simulink library "actuators_lib"  (R2018b)
settings: Solver=VariableStepAuto  StartTime=0.0  StopTime=10.0  RelTol=1e-3
libraries: $bdroot x1
settings Model: Creator=Ybeyer  LastModifiedBy=yannic
settings DebuggingCC: LibraryContextMissingDiagnostic=none
settings SFSimCC: SimUseLocalCustomCode=off
settings RTWCC: RTWUseLocalCustomCode=off
settings CodeAppCC: StateflowObjectComments=on

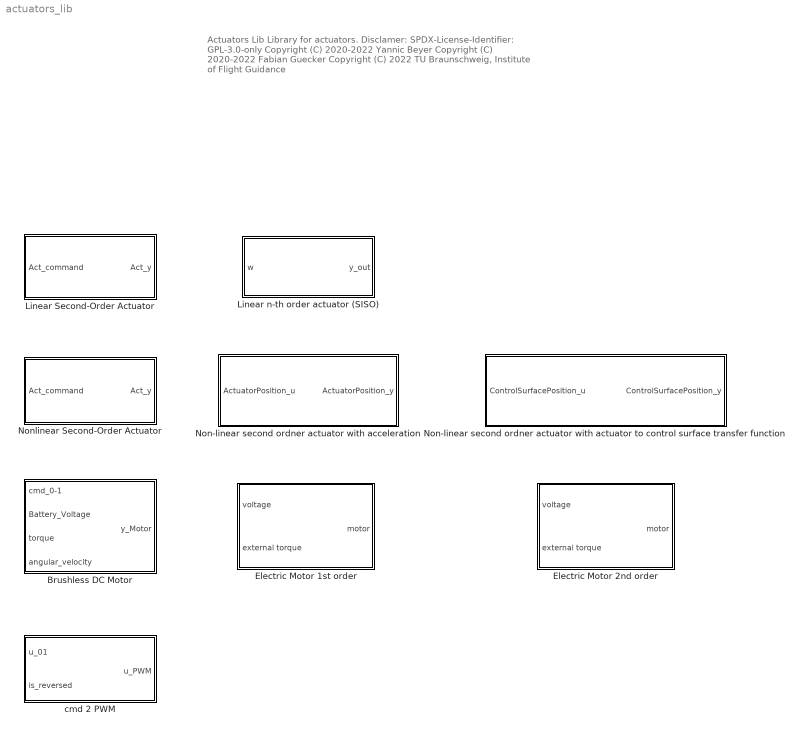
== system actuators_lib ==
  note: Actuators Lib
      |
      | Library for actuators.
      |
      | Disclamer:
      | SPDX-License-Identifier: GPL-3.0-only
      |
      | Copyright (C) 2020-2022 Yannic Beyer
      | Copyright (C) 2020-2022 Fabian Guecker
      | Copyright (C) 2022 TU Braunschweig, Institute of Flight Guidance
  Brushless DC Motor : Subsystem  mask{K_T=30/pi/920, J_prop=1e-04, R_i=0.042, IC_omega=0, omega_max=Inf, omega_min=0}
      mask prompts: K_T "Motor torque constant, Nm/A"; J_prop "Motor moment of inertia, kg-m^2"; R_i "Motor internal resistance, Ohm"; IC_omega "Initial motor angular velocity, 1/s"; omega_max "Maximum motor angular velocity, 1/s"; omega_min "Minimum motor angular velocity, 1/s"
      mask DialogControl DescGroupVar Prompt: Brushless DC Motor
      mask DialogControl DescTextVar Prompt: First-Order Brushless Direct Current Motor model.
      mask DialogControl Control3 Prompt: Inputs:
      mask DialogControl Control4 Prompt: Command (cmd_0-1, -)
      mask DialogControl Control5 Prompt: Battery Voltage, V
      mask DialogControl Control6 Prompt: torque, Nm
      mask DialogControl Control8 Prompt: Outputs:
      mask DialogControl Control9 Prompt: angular velocity (omega, 1/s)
      mask DialogControl Control10 Prompt: angular acceleration (dot_omega, 1/s^2)
  Electric Motor 1st order : Subsystem  mask{K_T=30/pi/920, J_prop=1e-04, R_i=0.042, IC_omega=0, omega_max=Inf, omega_min=0}
      mask prompts: K_T "Motor torque constant, Nm/A"; J_prop "Motor moment of inertia, kg-m^2"; R_i "Motor internal resistance, Ohm"; IC_omega "Initial motor angular velocity, rad/s"; omega_max "Maximum motor angular velocity, rad/s"; omega_min "Minimum motor angular velocity, rad/s"
      mask DialogControl DescGroupVar Prompt: Brushless DC Motor
      mask DialogControl DescTextVar Prompt: First-Order Brushless Direct Current Motor model.
      mask DialogControl Control3 Prompt: Inputs:
      mask DialogControl Control5 Prompt: - Supply Voltage, V
      mask DialogControl Control6 Prompt: - torque, Nm
  Electric Motor 2nd order : Subsystem  mask{K_T=30/pi/920, J_prop=1e-04, R_i=0.042, IC_omega=0, omega_max=Inf, omega_min=0, L=0}
      mask prompts: K_T "Motor torque constant, Nm/A"; J_prop "Motor moment of inertia, kg-m^2"; R_i "Motor internal resistance, Ohm"; IC_omega "Initial motor angular velocity, rad/s"; omega_max "Maximum motor angular velocity, rad/s"; omega_min "Minimum motor angular velocity, rad/s"; L "Motor inductance, H"
      mask DialogControl DescGroupVar Prompt: Brushless DC Motor
      mask DialogControl DescTextVar Prompt: First-Order Brushless Direct Current Motor model.
      mask DialogControl Control3 Prompt: Inputs:
      mask DialogControl Control5 Prompt: - Supply Voltage, V
      mask DialogControl Control6 Prompt: - torque, Nm
  Linear Second-Order Actuator : Subsystem  mask{omega=10, d=1, A_0=0, dot_A_0=0, start_steady_state=off}
      mask prompts: omega "Natural frequency"; d "Damping ratio"; A_0 "Initial position"; dot_A_0 "Initial velocity"; start_steady_state "Start steady state"
  Linear n-th order actuator (SISO) : Subsystem  mask{omega=10, order=5, output_order=6, use_inital_value=on}
      mask prompts: omega "Filter omega"; order "Filter order"; output_order "Output selection (max. order+1)"; use_inital_value "Start steady-state"
      mask init:
      | ss_model.order = order;
      | ss_model.omega = omega;
      | 
      | ss_model.K = ndiFeedbackGainPlace( -ss_model.omega*ones(ss_model.order,1), 0);
      | ss_model.A = diag(ones(ss_model.order-1,1),1);
      | ss_model.A(ss_model.order,:) = -ss_model.K';
      | 
      | ss_model.B = zeros(ss_model.order);
      | ss_model.C = eye(ss_model.order);
      | ss_model.D = zeros(ss_model.order);
      | 
      | ss_model.B(ss_model.order,ss_model.order) = ss_model.K(1);
  Non-linear second ordner actuator with acceleration : Subsystem  mask{omega=88, zeta=1, L1_pos=60, L1_neg=-60, L3_pos=753, L3_neg=-753, L2_pos=25440, L2_neg=-25440, inital_position=0, inital_velocity=0, dead_time=5.4 / 1000}
      mask prompts: omega "Natural frequency"; zeta "Damping ratio"; L1_pos "Maximum deflection"; L1_neg "Minimum deflection"; L3_pos "Maximum Rate"; L3_neg "Minimum Rate"; L2_pos "Maximum acceleration"; L2_neg "Minimum acceleration"; inital_position "Inital Position"; inital_velocity "Inital veloctiy"; dead_time "Dead time"
  Non-linear second ordner actuator with actuator to control surface transfer function : Subsystem  mask{ActuatorRefPosition=[-100 100], ControlSurfaceRefPosition=[-100 100], dead_time=5.4 / 1000, omega=88, zeta=1, L1_pos=+60, L1_neg=-60, L3_pos=753, L3_neg=-753, L2_pos=25440, L2_neg=-25440, inital_position=0, inital_velocity=0}
      mask prompts: ActuatorRefPosition "Actuator Position"; ControlSurfaceRefPosition "Control Surface Position"; dead_time "Dead time"; omega "Natural frequency"; zeta "Damping ratio"; L1_pos "Maximum deflection"; L1_neg "Minimum deflection"; L3_pos "Maximum Rate"; L3_neg "Minimum Rate"; L2_pos "Maximum acceleration"; L2_neg "Minimum acceleration"; inital_position "Inital Position"; inital_velocity "Inital veloctiy"
      mask TypeOptions dead_time: Subsystem/dead_time
      mask TypeOptions omega: Subsystem/omega
      mask TypeOptions zeta: Subsystem/zeta
      mask TypeOptions L1_pos: Subsystem/L1_pos
      mask TypeOptions L1_neg: Subsystem/L1_neg
      mask TypeOptions L3_pos: Subsystem/L3_pos
      mask TypeOptions L3_neg: Subsystem/L3_neg
      mask TypeOptions L2_pos: Subsystem/L2_pos
      mask TypeOptions L2_neg: Subsystem/L2_neg
      mask TypeOptions inital_position: Subsystem/inital_position
      mask TypeOptions inital_velocity: Subsystem/inital_velocity
      mask DialogControl Container3 Prompt: Transfer function from actuator position to control surface position
      mask DialogControl ParameterGroupVar Prompt: Actuator Parameters
  Nonlinear Second-Order Actuator : Subsystem  mask{omega=10, d=0.7, A_max=20*pi/180, A_min=-20*pi/180, dot_A_max=60*pi/180, dot_A_min=-60*pi/180, A_0=0, dot_A_0=0}
      mask prompts: omega "Natural frequency"; d "Damping ratio"; A_max "Maximum deflection"; A_min "Minimum deflection"; dot_A_max "Maximum rate"; dot_A_min "Minimum rate"; A_0 "Initial position"; dot_A_0 "Initial velocity"
  cmd 2 PWM : MATLAB Function  TreatAsAtomicUnit=on

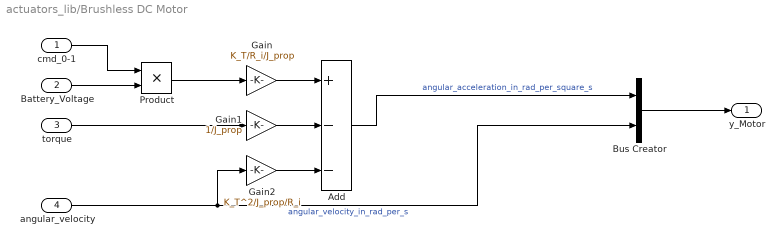
== system actuators_lib/Brushless DC Motor ==
  cmd_0-1 : Inport
  Battery_Voltage : Inport  Port=2
  torque : Inport  Port=3
  angular_velocity : Inport  Port=4
  Add : Sum  Inputs=+--
  Bus Creator : BusCreator  Inputs=2
  Gain : Gain  Gain=K_T/R_i/J_prop
  Gain1 : Gain  Gain=1/J_prop
  Gain2 : Gain  Gain=K_T^2/J_prop/R_i
  Product : Product
  y_Motor : Outport
  wires:
  Product/1 -> Gain/1
  torque/1 -> Gain1/1
  Gain1/1 -> Add/2
  angular_velocity/1 -> Bus Creator/2, Gain2/1  "angular_velocity_in_rad_per_s"
  Gain/1 -> Add/1
  Gain2/1 -> Add/3
  Add/1 -> Bus Creator/1  "angular_acceleration_in_rad_per_square_s"
  Battery_Voltage/1 -> Product/2
  cmd_0-1/1 -> Product/1
  Bus Creator/1 -> y_Motor/1

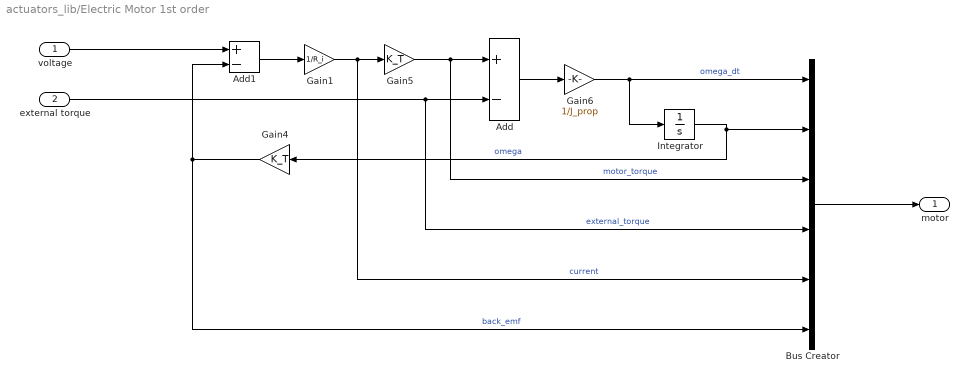
== system actuators_lib/Electric Motor 1st order ==
  voltage : Inport
  external torque : Inport  Port=2
  Add : Sum  Inputs=+-
  Add1 : Sum  Inputs=+-
  Bus Creator : BusCreator  Inputs=6
  Gain1 : Gain  Gain=1/R_i
  Gain4 : Gain  Gain=K_T
  Gain5 : Gain  Gain=K_T
  Gain6 : Gain  Gain=1/J_prop
  Integrator : Integrator  InitialCondition=IC_omega  LimitOutput=on  UpperSaturationLimit=omega_max  LowerSaturationLimit=omega_min
  motor : Outport
  wires:
  Bus Creator/1 -> motor/1
  Add/1 -> Gain6/1
  Add1/1 -> Gain1/1
  Integrator/1 -> Bus Creator/2, Gain4/1  "omega"
  external torque/1 -> Add/2, Bus Creator/4  "external_torque"
  voltage/1 -> Add1/1
  Gain6/1 -> Integrator/1, Bus Creator/1  "omega_dt"
  Gain1/1 -> Bus Creator/5, Gain5/1  "current"
  Gain4/1 -> Add1/2, Bus Creator/6  "back_emf"
  Gain5/1 -> Add/1, Bus Creator/3  "motor_torque"

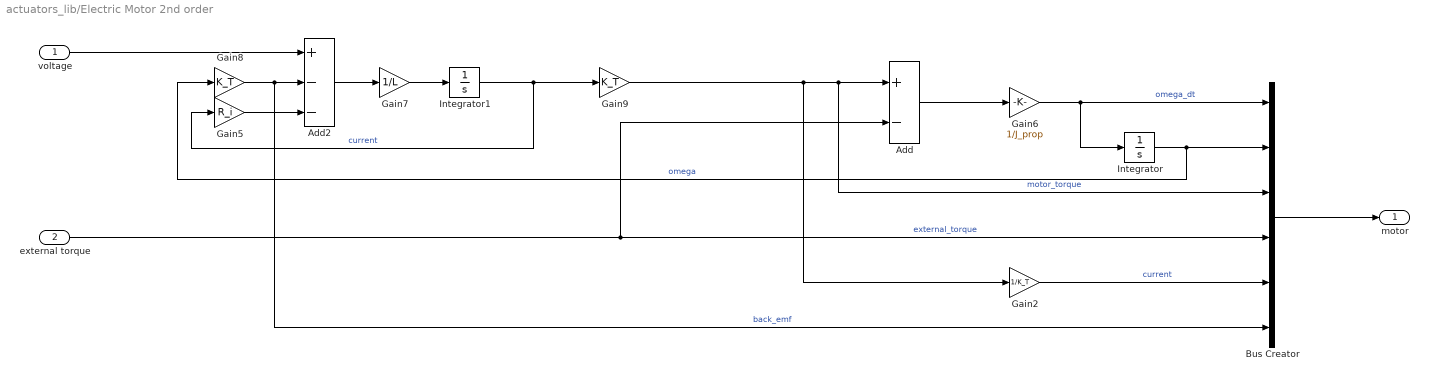
== system actuators_lib/Electric Motor 2nd order ==
  voltage : Inport
  external torque : Inport  Port=2
  Add : Sum  Inputs=+-
  Add2 : Sum  Inputs=+--
  Bus Creator : BusCreator  Inputs=6
  Gain2 : Gain  Gain=1/K_T
  Gain5 : Gain  Gain=R_i
  Gain6 : Gain  Gain=1/J_prop
  Gain7 : Gain  Gain=1/L
  Gain8 : Gain  Gain=K_T
  Gain9 : Gain  Gain=K_T
  Integrator : Integrator  InitialCondition=IC_omega  LimitOutput=on  UpperSaturationLimit=omega_max  LowerSaturationLimit=omega_min
  Integrator1 : Integrator
  motor : Outport
  wires:
  Gain2/1 -> Bus Creator/5  "current"
  Gain6/1 -> Integrator/1, Bus Creator/1  "omega_dt"
  voltage/1 -> Add2/1
  external torque/1 -> Add/2, Bus Creator/4  "external_torque"
  Integrator/1 -> Bus Creator/2, Gain8/1  "omega"
  Gain9/1 -> Add/1, Bus Creator/3, Gain2/1  "motor_torque"
  Add/1 -> Gain6/1
  Bus Creator/1 -> motor/1
  Integrator1/1 -> Gain9/1, Gain5/1  "current"
  Add2/1 -> Gain7/1
  Gain5/1 -> Add2/3
  Gain7/1 -> Integrator1/1
  Gain8/1 -> Bus Creator/6, Add2/2  "back_emf"

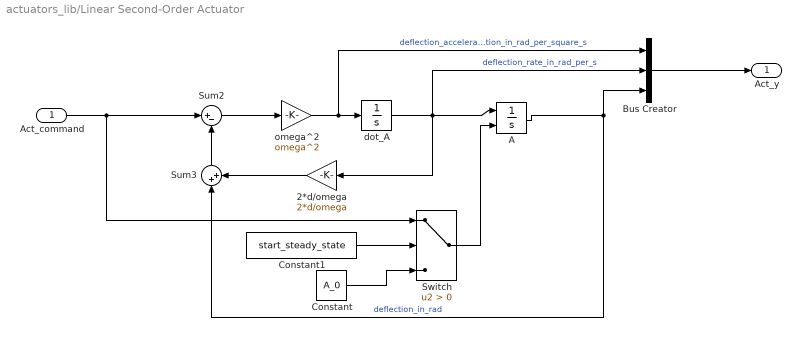
== system actuators_lib/Linear Second-Order Actuator ==
  Act_command : Inport
  2*d/omega : Gain  Gain=2*d/omega
  A : Integrator  InitialConditionSource=external  InitialCondition=A_0  ContinuousStateAttributes='A'
  Bus Creator : BusCreator  Inputs=3
  Constant : Constant  Value=A_0
  Constant1 : Constant  Value=start_steady_state
  Sum2 : Sum  Inputs=|+-
  Sum3 : Sum  Inputs=|++
  Switch : Switch  Criteria=u2 > Threshold  ZeroCross=off
  dot_A : Integrator  InitialCondition=dot_A_0  ContinuousStateAttributes='dot_A'
  omega^2 : Gain  Gain=omega^2
  Act_y : Outport
  wires:
  2*d/omega/1 -> Sum3/2
  dot_A/1 -> 2*d/omega/1, Bus Creator/2, A/1  "deflection_rate_in_rad_per_s"
  Act_command/1 -> Switch/1, Sum2/1
  Sum2/1 -> omega^2/1
  A/1 -> Bus Creator/3, Sum3/1  "deflection_in_rad"
  Sum3/1 -> Sum2/2
  omega^2/1 -> Bus Creator/1, dot_A/1  "deflection_acceleration_in_rad_per_square_s"
  Bus Creator/1 -> Act_y/1
  Switch/1 -> A/2
  Constant1/1 -> Switch/2
  Constant/1 -> Switch/3

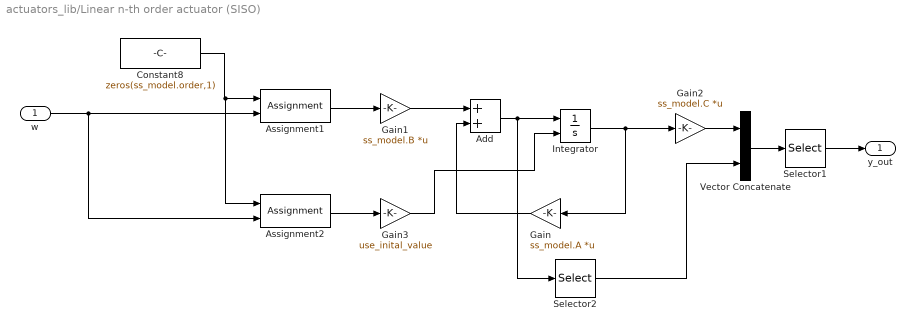
== system actuators_lib/Linear n-th order actuator (SISO) ==
  w : Inport
  Add : Sum
  Assignment1 : Assignment  DiagnosticForDimensions=Warning  IndexOptions=Index vector (dialog)  Indices=ss_model.order  OutputSizes=1
  Assignment2 : Assignment  DiagnosticForDimensions=Warning  IndexOptions=Index vector (dialog)  Indices=1  OutputSizes=1
  Constant8 : Constant  Value=zeros(ss_model.order,1)  VectorParams1D=off
  Gain : Gain  Gain=ss_model.A  Multiplication=Matrix(K*u)
  Gain1 : Gain  Gain=ss_model.B  Multiplication=Matrix(K*u)
  Gain2 : Gain  Gain=ss_model.C  Multiplication=Matrix(K*u)
  Gain3 : Gain  Gain=use_inital_value
  Integrator : Integrator  InitialConditionSource=external
  Selector1 : Selector  InputPortWidth=ss_model.order+1  IndexOptions=Index vector (dialog)  Indices=1:min(output_order, ss_model.order+1)  OutputSizes=1
  Selector2 : Selector  InputPortWidth=ss_model.order  IndexOptions=Index vector (dialog)  Indices=ss_model.order  OutputSizes=1
  Vector Concatenate : Concatenate
  y_out : Outport
  wires:
  Constant8/1 -> Assignment2/1, Assignment1/1
  w/1 -> Assignment2/2, Assignment1/2
  Integrator/1 -> Gain2/1, Gain/1
  Gain1/1 -> Add/1
  Assignment1/1 -> Gain1/1
  Add/1 -> Selector2/1, Integrator/1
  Gain2/1 -> Vector Concatenate/1
  Gain/1 -> Add/2
  Assignment2/1 -> Gain3/1
  Gain3/1 -> Integrator/2
  Selector1/1 -> y_out/1
  Selector2/1 -> Vector Concatenate/2
  Vector Concatenate/1 -> Selector1/1

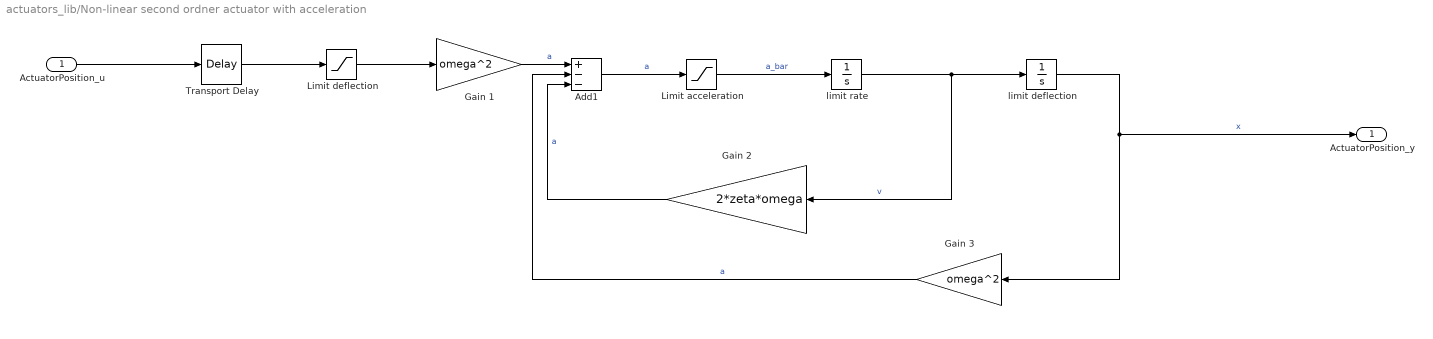
== system actuators_lib/Non-linear second ordner actuator with acceleration ==
  ActuatorPosition_u : Inport
  Add1 : Sum  Inputs=+--
  Gain 1 : Gain  Gain=omega^2
  Gain 2 : Gain  Gain=2*zeta*omega
  Gain 3 : Gain  Gain=omega^2
  Limit acceleration : Saturate  UpperLimit=L2_pos  LowerLimit=L2_neg
  Limit deflection : Saturate  UpperLimit=L1_pos  LowerLimit=L1_neg
  Transport Delay : TransportDelay  DelayTime=dead_time  InitialOutput=inital_position
  limit deflection : Integrator  InitialCondition=inital_position  LimitOutput=on  UpperSaturationLimit=L1_pos  LowerSaturationLimit=L1_neg
  limit rate : Integrator  InitialCondition=inital_velocity  LimitOutput=on  UpperSaturationLimit=L3_pos  LowerSaturationLimit=L3_neg
  ActuatorPosition_y : Outport  VectorParamsAs1DForOutWhenUnconnected=on
  wires:
  Limit deflection/1 -> Gain 1/1
  Transport Delay/1 -> Limit deflection/1
  Gain 2/1 -> Add1/3  "a"
  Add1/1 -> Limit acceleration/1  "a"
  Gain 3/1 -> Add1/2  "a"
  Gain 1/1 -> Add1/1  "a"
  ActuatorPosition_u/1 -> Transport Delay/1
  Limit acceleration/1 -> limit rate/1  "a_bar"
  limit rate/1 -> limit deflection/1, Gain 2/1  "v"
  limit deflection/1 -> ActuatorPosition_y/1, Gain 3/1  "x"

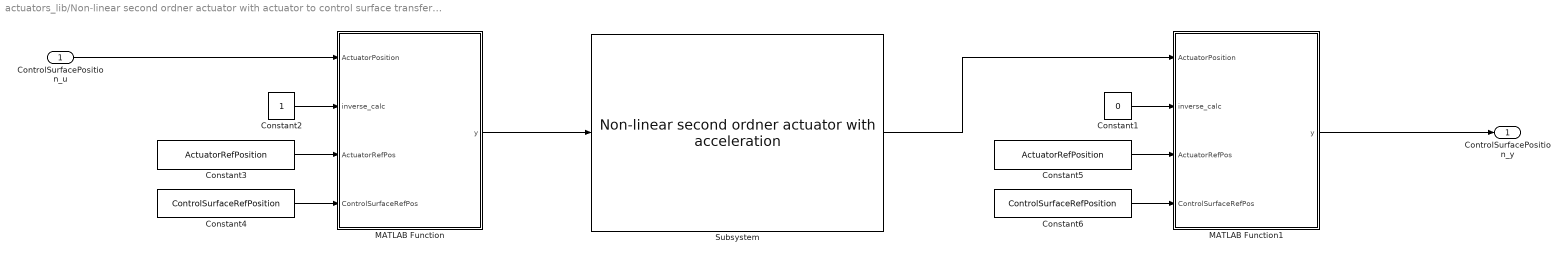
== system actuators_lib/Non-linear second ordner actuator with actuator to control surface transfer function ==
  ControlSurfacePosition_u : Inport
  Constant1 : Constant  Value=0
  Constant2 : Constant
  Constant3 : Constant  Value=ActuatorRefPosition
  Constant4 : Constant  Value=ControlSurfaceRefPosition
  Constant5 : Constant  Value=ActuatorRefPosition
  Constant6 : Constant  Value=ControlSurfaceRefPosition
  MATLAB Function : MATLAB Function  TreatAsAtomicUnit=on
  MATLAB Function1 : MATLAB Function  TreatAsAtomicUnit=on
  Subsystem : $bdroot/Non-linear second ordner actuator with acceleration  omega=omega  zeta=zeta  L1_pos=L1_pos  L1_neg=L1_neg  L3_pos=L3_pos  L3_neg=L3_neg  L2_pos=L2_pos  L2_neg=L2_neg  inital_position=inital_position  inital_velocity=inital_velocity  dead_time=dead_time
  ControlSurfacePosition_y : Outport  VectorParamsAs1DForOutWhenUnconnected=on
  wires:
  Constant2/1 -> MATLAB Function/2(inverse_calc)
  Constant6/1 -> MATLAB Function1/4(ControlSurfaceRefPos)
  ControlSurfacePosition_u/1 -> MATLAB Function/1(ActuatorPosition)
  MATLAB Function/1(y) -> Subsystem/1
  Constant1/1 -> MATLAB Function1/2(inverse_calc)
  MATLAB Function1/1(y) -> ControlSurfacePosition_y/1
  Constant4/1 -> MATLAB Function/4(ControlSurfaceRefPos)
  Subsystem/1 -> MATLAB Function1/1(ActuatorPosition)
  Constant3/1 -> MATLAB Function/3(ActuatorRefPos)
  Constant5/1 -> MATLAB Function1/3(ActuatorRefPos)

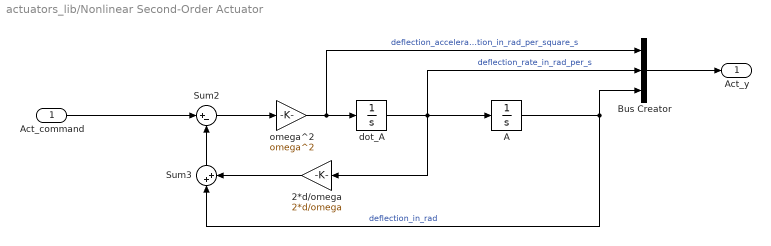
== system actuators_lib/Nonlinear Second-Order Actuator ==
  Act_command : Inport
  2*d/omega : Gain  Gain=2*d/omega
  A : Integrator  InitialCondition=A_0  LimitOutput=on  UpperSaturationLimit=A_max  LowerSaturationLimit=A_min  ContinuousStateAttributes='A'
  Bus Creator : BusCreator  Inputs=3
  Sum2 : Sum  Inputs=|+-
  Sum3 : Sum  Inputs=|++
  dot_A : Integrator  InitialCondition=dot_A_0  LimitOutput=on  UpperSaturationLimit=dot_A_max  LowerSaturationLimit=dot_A_min  ContinuousStateAttributes='dot_A'
  omega^2 : Gain  Gain=omega^2
  Act_y : Outport
  wires:
  A/1 -> Bus Creator/3, Sum3/1  "deflection_in_rad"
  dot_A/1 -> Bus Creator/2, 2*d/omega/1, A/1  "deflection_rate_in_rad_per_s"
  Act_command/1 -> Sum2/1
  Sum3/1 -> Sum2/2
  2*d/omega/1 -> Sum3/2
  Sum2/1 -> omega^2/1
  omega^2/1 -> Bus Creator/1, dot_A/1  "deflection_acceleration_in_rad_per_square_s"
  Bus Creator/1 -> Act_y/1

== matlab function actuators_lib/Non-linear second ordner actuator with actuator to control surface transfer function/MATLAB Function ==
  data: ActuatorPosition input; y output; inverse_calc input; ActuatorRefPos input; ControlSurfaceRefPos input
function y = fcn(ActuatorPosition, inverse_calc, ActuatorRefPos, ControlSurfaceRefPos)

y = mapActuatorToControlSurface(ActuatorPosition, inverse_calc, ActuatorRefPos, ControlSurfaceRefPos);

== matlab function actuators_lib/cmd 2 PWM ==
  data: u_01 input; u_PWM output; is_reversed input
function u_PWM = fcn(u_01,is_reversed) %codegen
    u_PWM = cmd2PWM(u_01,is_reversed);
end

== matlab function actuators_lib/Non-linear second ordner actuator with actuator to control surface transfer function/MATLAB Function1 ==
  data: ActuatorPosition input; y output; inverse_calc input; ActuatorRefPos input; ControlSurfaceRefPos input
function y = fcn(ActuatorPosition, inverse_calc, ActuatorRefPos, ControlSurfaceRefPos)

y = mapActuatorToControlSurface(ActuatorPosition, inverse_calc, ActuatorRefPos, ControlSurfaceRefPos);
